simulink model "StateControl"  (R2023b)
settings: Solver=FixedStepDiscrete  StartTime=0.0  StopTime=10.0  FixedStep=1e-4  RelTol=1e-3
settings Model: DataDictionary=StateControl.sldd  Creator=84339  LastModifiedBy=84339
settings OptimizationCC: DefaultParameterBehavior=Inlined  EnhancedBackFolding=on  PassReuseOutputArgsAs=Individual arguments  ZeroExternalMemoryAtStartup=off  ZeroInternalMemoryAtStartup=off  OptimizeBlockOrder=speed  DifferentSizesBufferReuse=on  OptimizationCustomize=off  EfficientTunableParamExpr=on
settings DebuggingCC: ParameterTunabilityLossMsg=error
settings SFSimCC: MATLABDynamicMemAlloc=off
settings RTWCC: Description=Embedded Coder  SystemTargetFile=ert.tlc  EmbeddedCoderDictionary=Arch.sldd  GenCodeOnly=on  TemplateMakefile=ert_default_tmf
settings CodeAppCC: ForceParamTrailComments=on  IgnoreCustomStorageClasses=off  OperatorAnnotations=on  SimulinkDataObjDesc=on  SFDataObjDesc=on  InsertBlockDesc=on
settings ERTTargetCC: TargetLangStandard=C99 (ISO)  GenerateSampleERTMain=on  InlinedParameterPlacement=NonHierarchical  ERTCustomFileTemplate=example_file_process.tlc

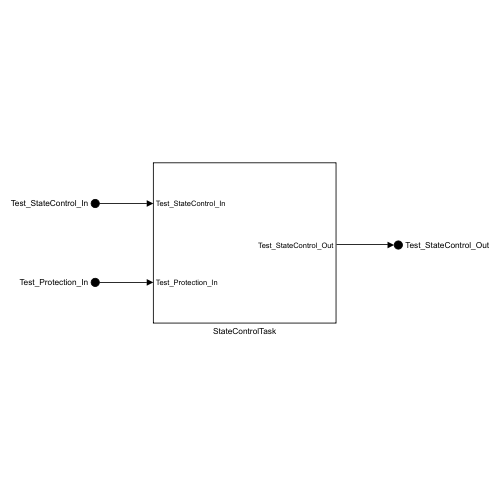
[thumbnail: Simulink's stored preview of the top-level diagram]
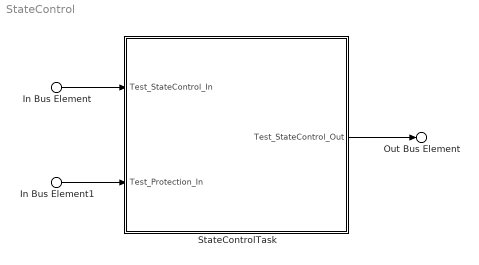
== system StateControl ==
  In Bus Element : Inport  PortName=Test_StateControl_In
  In Bus Element1 : Inport  Port=2  PortName=Test_Protection_In
  StateControlTask : Subsystem
  Out Bus Element : Outport  PortName=Test_StateControl_Out
  wires:
  In Bus Element/1 -> StateControlTask/1(Test_StateControl_In)
  StateControlTask/1(Test_StateControl_Out) -> Out Bus Element/1
  In Bus Element1/1 -> StateControlTask/2(Test_Protection_In)

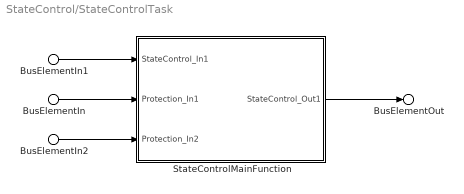
== system StateControl/StateControlTask ==
  BusElementIn1 : Inport  PortName=Test_StateControl_In  Element=StateControl_In1
  BusElementIn : Inport  Port=2  PortName=Test_Protection_In  Element=Protection_In1
  BusElementIn2 : Inport  Port=2  PortName=Test_Protection_In  Element=Protection_In2
  StateControlMainFunction : Subsystem
  BusElementOut : Outport  PortName=Test_StateControl_Out  Element=StateControl_Out1
  wires:
  BusElementIn1/1 -> StateControlMainFunction/1(StateControl_In1)
  StateControlMainFunction/1(StateControl_Out1) -> BusElementOut/1
  BusElementIn/1 -> StateControlMainFunction/2(Protection_In1)
  BusElementIn2/1 -> StateControlMainFunction/3(Protection_In2)

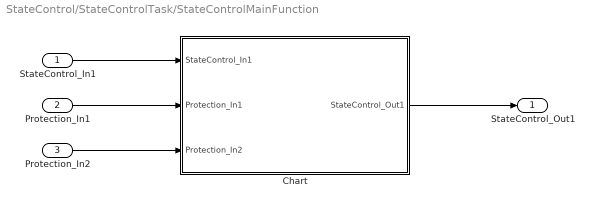
== system StateControl/StateControlTask/StateControlMainFunction ==
  StateControl_In1 : Inport
  Protection_In1 : Inport  Port=2
  Protection_In2 : Inport  Port=3
  Chart : Stateflow chart  TreatAsAtomicUnit=on
  StateControl_Out1 : Outport
  wires:
  Chart/1(StateControl_Out1) -> StateControl_Out1/1
  StateControl_In1/1 -> Chart/1(StateControl_In1)
  Protection_In1/1 -> Chart/2(Protection_In1)
  Protection_In2/1 -> Chart/3(Protection_In2)

== stateflow chart StateControl/StateControlTask/StateControlMainFunction/Chart ==
  state Off1
    en:
    StateControl_Out1 = STCTL_MODE_CONTROL.OFF;
  state On
    en:
    StateControl_Out1 = STCTL_MODE_CONTROL.ON
  (default) -> Off1
  Off1 -> On : [(StateControl_In1 == STCTL_MODE_CONTROL.ON) && (Protection_In1 >= Protection_In2) && (Protection_In2 >= 400)]
  On -> Off1 : [StateControl_In1 == STCTL_MODE_CONTROL.OFF]
  data: StateControl_In1 input; Protection_In1 input; Protection_In2 input; StateControl_Out1 output
